simulink model "lab4_1"  (R2025b)
settings: Solver=VariableStepAuto  StartTime=0.0  StopTime=10.0  RelTol=1e-3
undefined symbols (not defined in the file): A_M, b, b_M, disturbance_on, gamma, kappa, P, sigma
settings Model: Creator=Nickolay  LastModifiedBy=Nickolay

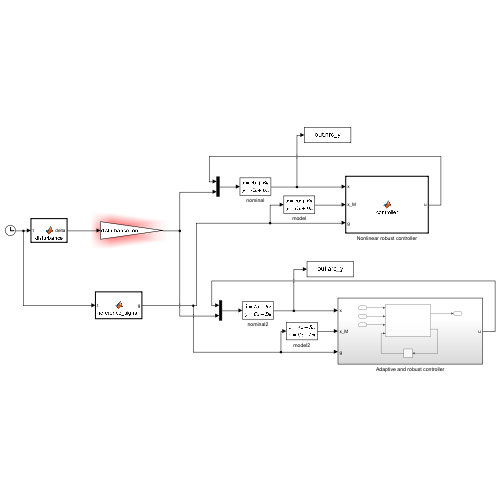
[thumbnail: Simulink's stored preview of the top-level diagram]
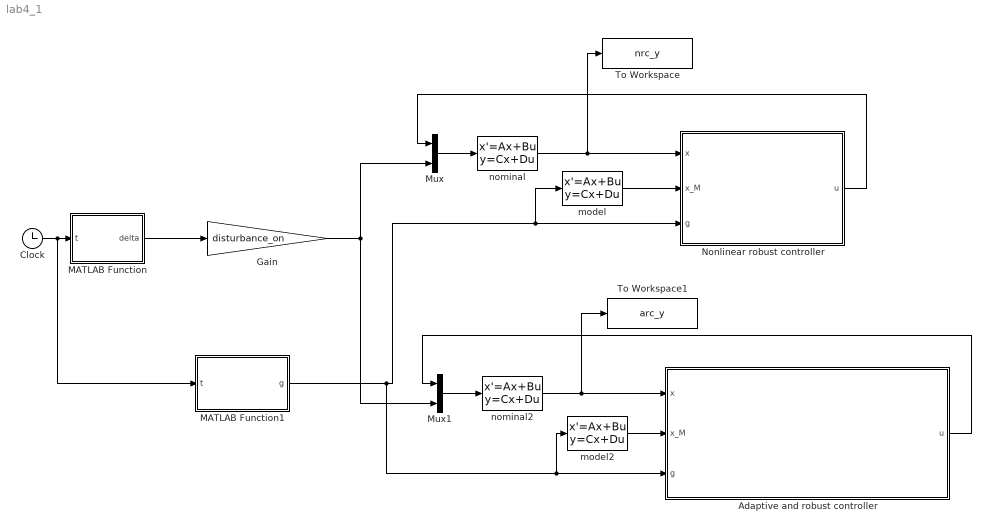
== system lab4_1 ==
  Adaptive and robust controller : Subsystem
  Clock : Clock
  Gain : Gain  Gain=disturbance_on
  MATLAB Function : MATLAB Function  TreatAsAtomicUnit=on
  MATLAB Function1 : MATLAB Function  TreatAsAtomicUnit=on
  Mux : Mux  Inputs=2
  Mux1 : Mux  Inputs=2
  Nonlinear robust controller : MATLAB Function  TreatAsAtomicUnit=on
  To Workspace : ToWorkspace  VariableName=nrc_y  SaveFormat=Timeseries  SampleTime=-1
  To Workspace1 : ToWorkspace  VariableName=arc_y  SaveFormat=Timeseries  SampleTime=-1
  model : StateSpace  A=A_M  B=b_M  C=eye(2)  D=zeros(2,1)  InitialCondition=[0; 0]
  model2 : StateSpace  A=A_M  B=b_M  C=eye(2)  D=zeros(2,1)  InitialCondition=[0; 0]
  nominal : StateSpace  A=[0 1; 1 1]  B=[b eye(2)]  C=eye(2)  D=zeros(2, 3)  InitialCondition=[0; 0]
  nominal2 : StateSpace  A=[0 1; 1 1]  B=[b eye(2)]  C=eye(2)  D=zeros(2, 3)  InitialCondition=[0; 0]
  wires:
  Clock/1 -> MATLAB Function1/1(t), MATLAB Function/1(t)
  Nonlinear robust controller/1(u) -> Mux/1
  Mux/1 -> nominal/1
  Mux1/1 -> nominal2/1
  Adaptive and robust controller/1(u) -> Mux1/1
  nominal/1 -> To Workspace/1, Nonlinear robust controller/1(x)
  nominal2/1 -> To Workspace1/1, Adaptive and robust controller/1(x)
  model/1 -> Nonlinear robust controller/2(x_M)
  model2/1 -> Adaptive and robust controller/2(x_M)
  MATLAB Function1/1(g) -> model2/1, Adaptive and robust controller/3(g), model/1, Nonlinear robust controller/3(g)
  Gain/1 -> Mux1/2, Mux/2
  MATLAB Function/1(delta) -> Gain/1

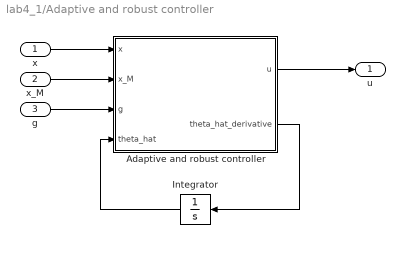
== system lab4_1/Adaptive and robust controller ==
  x : Inport
  x_M : Inport  Port=2
  g : Inport  Port=3
  Adaptive and robust controller : MATLAB Function  TreatAsAtomicUnit=on
  Integrator : Integrator
  u : Outport
  wires:
  x/1 -> Adaptive and robust controller/1(x)
  Adaptive and robust controller/2(theta_hat_derivative) -> Integrator/1
  Integrator/1 -> Adaptive and robust controller/4(theta_hat)
  Adaptive and robust controller/1(u) -> u/1
  x_M/1 -> Adaptive and robust controller/2(x_M)
  g/1 -> Adaptive and robust controller/3(g)

== matlab function lab4_1/MATLAB Function ==
  data: t input; delta output
function delta = disturbance(t)

delta = [
    0.6*sin(10*t) + 0.1*sin(50*t);
    0.5*cos(12*t) + 0.2*sin(30*t)
];

end

== matlab function lab4_1/Nonlinear robust controller ==
  data: x input; x_M input; u output; g input; b parameter; P parameter; gamma parameter; kappa parameter
function u = controller(x, x_M, g, b, P, gamma, kappa)
e = x_M - x;
theta_hat = gamma * x * b.' * P * e;
u = theta_hat.' * x + 1/kappa * g;
end

== matlab function lab4_1/Adaptive and robust controller/Adaptive and robust controller ==
  data: x input; x_M input; u output; g input; theta_hat_derivative output; b parameter; P parameter; gamma parameter; kappa parameter; theta_hat input; sigma parameter
function [u, theta_hat_derivative]= controller(x, x_M, g, b, P, gamma, kappa, theta_hat, sigma)
e = x_M - x;
theta_hat_derivative = gamma * x * b.' * P * e - sigma * theta_hat;
u = theta_hat.' * x + 1/kappa * g;
end

== matlab function lab4_1/MATLAB Function1 ==
  data: t input; g output
function g = reference_signal(t)

g = 3 * sign(cos(0.2 * t)) + 3;

end
